simulink library "Contact_Forces_Lib"  (R2025a)
settings: Solver=ode45  StartTime=0.0  StopTime=10.0  RelTol=1e-3  EnableMultiTasking=on
undefined symbols (not defined in the file or in its folder): b_contact, custom_param_1, custom_param_2, Extr_Data_Ring, k_contact, l_cone, length_cylinder, length_tube, mu_kinetic, mu_static, pen_exponent, pen_full_damp_F, rad_s_cone, radius_cylinder, radius_tube, v_thr, X, Y, Z
libraries: nesl_utility x197, sm_lib x115, $bdroot x72, simulink x20, fl_lib x4
(part 12 of 12)

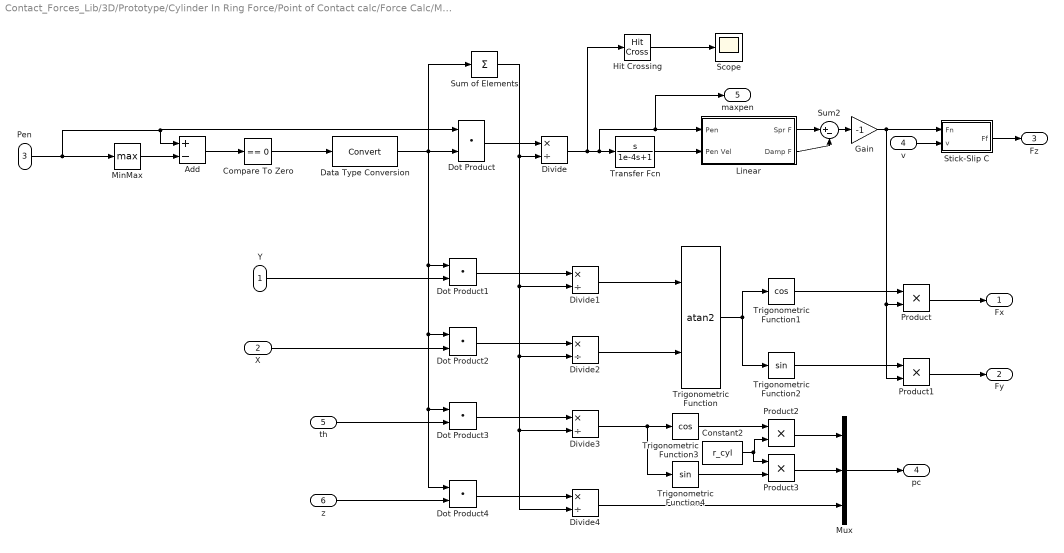
== system Contact_Forces_Lib/3D/Prototype/Cylinder In Ring Force/Point of Contact calc/Force Calc/MAX_SL ==
  Y : Inport
  X : Inport  Port=2
  Pen : Inport  Port=3
  v : Inport  Port=4
  th : Inport  Port=5
  z : Inport  Port=6
  Add : Sum  Inputs=+-
  Compare To Zero : simulink/Logic and Bit Operations/Compare To Zero  relop===  OutDataTypeStr=boolean  ZeroCross=off
  Constant2 : Constant  Value=r_cyl
  Data Type Conversion : DataTypeConversion  SaturateOnIntegerOverflow=off  RndMeth=Floor
  Divide{,1..4} (5 alike) : Product  Inputs=*/
  Dot Product{,1..4} (5 alike) : DotProduct  OutDataTypeStr=Inherit: Inherit via internal rule
  Gain : Gain  Gain=-1
  Hit Crossing : HitCross
  Linear : Subsystem  VariantControl=Linear  mask(Linear Force Law){k_pen=k_stiff, b_penvel=b_damp}
      mask prompts: k_pen "Contact Stiffness"; b_penvel "Contact Damping"
      mask help: Implements a contact force law as a linear spring damper. The damping force is applied only as the penetration depth increases.
      mask Help: web(which('Force_Laws.html'));
  MinMax : MinMax  Function=max  ZeroCross=off
  Mux : Mux  Inputs=3
  Product{,1..3} (4 alike) : Product
  Scope : Scope
      settings: DataLoggingVariableName=ScopeData3  DataLoggingSaveFormat=Array
  "Stick-Slip C " : Subsystem  VariantControl=Stick_Slip_C  mask(Stick-Slip Friction, Continuous){muk=mu_kinetic, mus=mu_static, vth=v_thr}
      mask prompts: muk "Coefficient of Kinetic Friction"; mus "Coefficient of Static Friction"; vth "Velocity Threshold"
      mask help: Implements a continuous stick-slip friction model. Smaller velocity threshold is closer to reality but results in a numerically stiffer system.
  Sum of Elements : Sum  Inputs=+
  Sum2 : Sum  Inputs=|+-
  Transfer Fcn : TransferFcn  Numerator=[1 0]  Denominator=[1e-4 1]
  Trigonometric Function : Trigonometry  Operator=atan2
  Trigonometric Function1 : Trigonometry  Operator=cos
  Trigonometric Function2 : Trigonometry
  Trigonometric Function3 : Trigonometry  Operator=cos
  Trigonometric Function4 : Trigonometry
  Fx : Outport  VectorParamsAs1DForOutWhenUnconnected=off
  Fy : Outport  Port=2  VectorParamsAs1DForOutWhenUnconnected=off
  Fz : Outport  Port=3  VectorParamsAs1DForOutWhenUnconnected=off
  pc : Outport  Port=4  VectorParamsAs1DForOutWhenUnconnected=off
  maxpen : Outport  Port=5  VectorParamsAs1DForOutWhenUnconnected=off
  wires:
  Trigonometric Function/1 -> Trigonometric Function2/1, Trigonometric Function1/1
  Linear/2(Damp F) -> Sum2/2
  Sum2/1 -> Gain/1
  Trigonometric Function2/1 -> Product1/1
  Linear/1(Spr F) -> Sum2/1
  Trigonometric Function1/1 -> Product/1
  Gain/1 -> "Stick-Slip C "/1(Fn), Product1/2, Product/2
  Transfer Fcn/1 -> Linear/2(Pen Vel)
  MinMax/1 -> Add/2
  Add/1 -> Compare To Zero/1
  Compare To Zero/1 -> Data Type Conversion/1
  Product/1 -> Fx/1
  Pen/1 -> Dot Product/1, Add/1, MinMax/1
  Product1/1 -> Fy/1
  Y/1 -> Dot Product1/2
  X/1 -> Dot Product2/2
  Data Type Conversion/1 -> Dot Product/2, Dot Product4/1, Dot Product3/1, Dot Product2/1, Dot Product1/1, Sum of Elements/1
  Dot Product/1 -> Divide/1
  Sum of Elements/1 -> Divide1/2, Divide4/2, Divide3/2, Divide2/2, Divide/2
  Divide/1 -> Hit Crossing/1, maxpen/1, Linear/1(Pen), Transfer Fcn/1
  Dot Product1/1 -> Divide1/1
  Dot Product2/1 -> Divide2/1
  Divide1/1 -> Trigonometric Function/1
  Divide2/1 -> Trigonometric Function/2
  Hit Crossing/1 -> Scope/1
  v/1 -> "Stick-Slip C "/2(v)
  Dot Product3/1 -> Divide3/1
  Dot Product4/1 -> Divide4/1
  th/1 -> Dot Product3/2
  z/1 -> Dot Product4/2
  Divide3/1 -> Trigonometric Function4/1, Trigonometric Function3/1
  Trigonometric Function3/1 -> Product2/1
  Trigonometric Function4/1 -> Product3/2
  Constant2/1 -> Product3/1, Product2/2
  Product2/1 -> Mux/1
  Product3/1 -> Mux/2
  Divide4/1 -> Mux/3
  "Stick-Slip C "/1(Ff) -> Fz/1
  Mux/1 -> pc/1

== system Contact_Forces_Lib/3D/Sphere to Cone Force/Forces/Ff/Relative vel at CP/Calculate vRelFace ==
  rSphtoCP sign : Inport
  azm : Inport  Port=2
  wxf : Inport  Port=3
  wyf : Inport  Port=4
  vzf : Inport  Port=5
  vrad : Inport  Port=6
  Gain : Gain  Gain=cosConeTh
  Gain{1..2,4..5} (4 alike) : Gain  Gain=-1
  Gain3 : Gain  Gain=sinConeTh
  Product : Product
  Product1 : Product
  Product2 : Product
  Sum : Sum
  Sum1 : Sum
  Sum3 : Sum
  Trigonometric Function3 : Trigonometry  Operator=cos
  Trigonometric Function4 : Trigonometry
  vRelFace : Outport  VectorParamsAs1DForOutWhenUnconnected=off
  wires:
  Gain4/1 -> Sum3/2  "vFaceTra"
  Gain5/1 -> Sum1/1
  Gain3/1 -> Gain5/1
  vzf/1 -> Gain3/1
  Gain/1 -> Sum1/2
  vrad/1 -> Gain/1
  Gain1/1 -> Product2/1
  Gain2/1 -> Sum/2  "wyCP"
  Trigonometric Function4/1 -> Product/1
  Product1/1 -> Gain2/1
  Sum3/1 -> vRelFace/1  "vRelFace"
  wyf/1 -> Product1/2
  Sum/1 -> Product2/2  "wxyzCP"
  rSphtoCP sign/1 -> Gain1/1
  Sum1/1 -> Gain4/1
  Product/1 -> Sum/1  "wxCP"
  wxf/1 -> Product/2
  Trigonometric Function3/1 -> Product1/1
  Product2/1 -> Sum3/1  "vFaceRot"
  azm/1 -> Trigonometric Function3/1, Trigonometric Function4/1

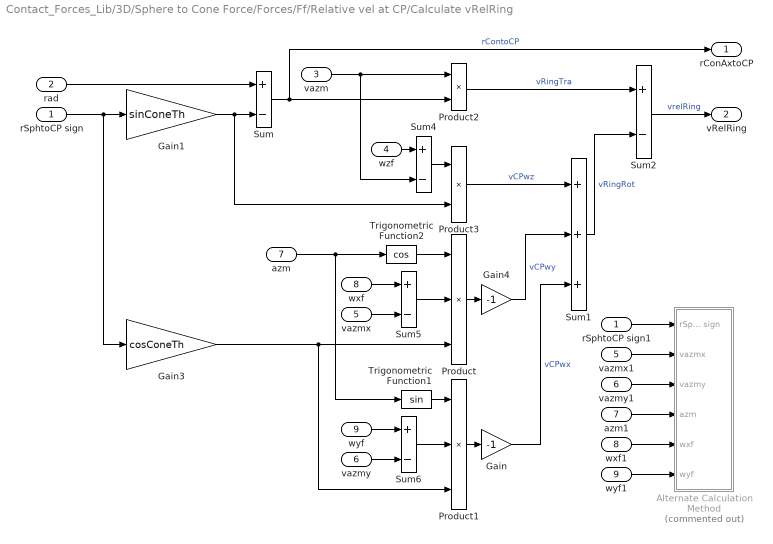
== system Contact_Forces_Lib/3D/Sphere to Cone Force/Forces/Ff/Relative vel at CP/Calculate vRelRing ==
  rSphtoCP sign : Inport
  rad : Inport  Port=2
  vazm : Inport  Port=3
  wzf : Inport  Port=4
  vazmx : Inport  Port=5
  vazmy : Inport  Port=6
  azm : Inport  Port=7
  wxf : Inport  Port=8
  wyf : Inport  Port=9
  Alternate Calculation Method : Subsystem  Commented=on
  Gain : Gain  Gain=-1
  Gain1 : Gain  Gain=sinConeTh
  Gain3 : Gain  Gain=cosConeTh
  Gain4 : Gain  Gain=-1
  Product : Product  Inputs=3
  Product1 : Product  Inputs=3
  Product2 : Product
  Product3 : Product
  Sum{,2,4..6} (5 alike) : Sum  Inputs=+-
  Sum1 : Sum  Inputs=+++
  Trigonometric Function1 : Trigonometry
  Trigonometric Function2 : Trigonometry  Operator=cos
  azm1 : InportShadow  Port=7
  rSphtoCP sign1 : InportShadow
  vazmx1 : InportShadow  Port=5
  vazmy1 : InportShadow  Port=6
  wxf1 : InportShadow  Port=8
  wyf1 : InportShadow  Port=9
  rConAxtoCP : Outport  VectorParamsAs1DForOutWhenUnconnected=off
  vRelRing : Outport  Port=2  VectorParamsAs1DForOutWhenUnconnected=off
  wires:
  wyf1/1 -> Alternate Calculation Method/6(wyf)
  wxf1/1 -> Alternate Calculation Method/5(wxf)
  azm1/1 -> Alternate Calculation Method/4(azm)
  vazmy1/1 -> Alternate Calculation Method/3(vazmy)
  vazmx1/1 -> Alternate Calculation Method/2(vazmx)
  rSphtoCP sign1/1 -> Alternate Calculation Method/1(rSphtoCP sign)
  Gain4/1 -> Sum1/2  "vCPwy"
  Sum6/1 -> Product1/2
  vazmy/1 -> Sum6/2
  wyf/1 -> Sum6/1
  vazmx/1 -> Sum5/2
  wxf/1 -> Sum5/1
  Product3/1 -> Sum1/1  "vCPwz"
  Gain3/1 -> Product1/3, Product/3
  Gain/1 -> Sum1/3  "vCPwx"
  Product1/1 -> Gain/1
  Trigonometric Function1/1 -> Product1/1
  Sum5/1 -> Product/2
  azm/1 -> Trigonometric Function1/1, Trigonometric Function2/1
  Product/1 -> Gain4/1
  Trigonometric Function2/1 -> Product/1
  Gain1/1 -> Sum/2, Product3/2
  rSphtoCP sign/1 -> Gain3/1, Gain1/1
  rad/1 -> Sum/1
  wzf/1 -> Sum4/1
  vazm/1 -> Product2/1, Sum4/2
  Product2/1 -> Sum2/1  "vRingTra"
  Sum/1 -> rConAxtoCP/1, Product2/2  "rContoCP"
  Sum2/1 -> vRelRing/1  "vrelRing"
  Sum1/1 -> Sum2/2  "vRingRot"
  Sum4/1 -> Product3/1

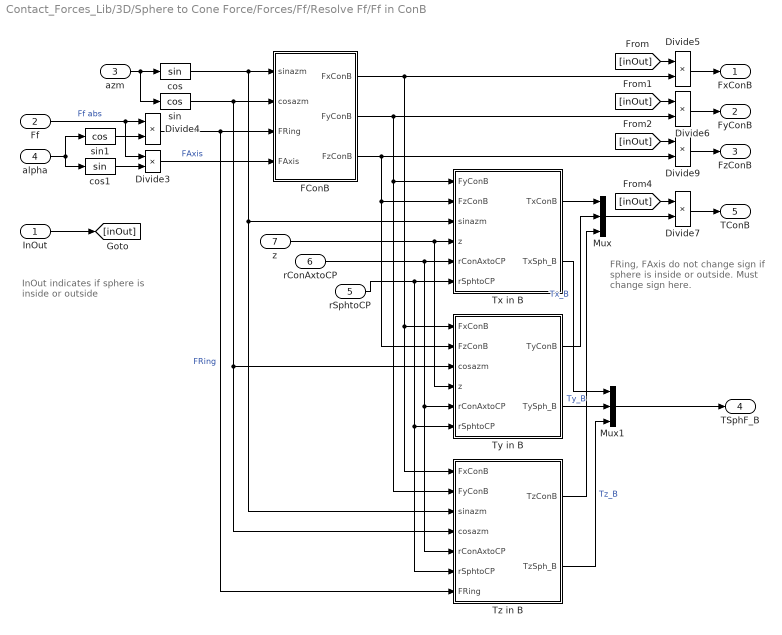
== system Contact_Forces_Lib/3D/Sphere to Cone Force/Forces/Ff/Resolve Ff/Ff in ConB ==
  note: InOut indicates if sphere is inside or outside
  note: FRing, FAxis do not change sign if sphere is inside or outside. Must change sign here.
  InOut : Inport
  Ff : Inport  Port=2
  azm : Inport  Port=3
  alpha : Inport  Port=4
  rSphtoCP : Inport  Port=5
  rConAxtoCP : Inport  Port=6
  z : Inport  Port=7
  Divide{3..7,9} (6 alike) : Product  Inputs=**
  FConB : Subsystem
  Mux : Mux  Inputs=3
  Mux1 : Mux  Inputs=3
  Tx in B : Subsystem
  Ty in B : Subsystem
  Tz in B : Subsystem
  cos : Trigonometry
  cos1 : Trigonometry
  sin : Trigonometry  Operator=cos
  sin1 : Trigonometry  Operator=cos
  FxConB : Outport  VectorParamsAs1DForOutWhenUnconnected=off
  FyConB : Outport  Port=2  VectorParamsAs1DForOutWhenUnconnected=off
  FzConB : Outport  Port=3  VectorParamsAs1DForOutWhenUnconnected=off
  TSphF_B : Outport  Port=4  VectorParamsAs1DForOutWhenUnconnected=off
  TConB : Outport  Port=5  VectorParamsAs1DForOutWhenUnconnected=off
  wires:
  FConB/2(FyConB) -> Divide6/2, Tz in B/2(FyConB), Tx in B/1(FyConB)
  Mux1/1 -> TSphF_B/1
  Divide3/1 -> FConB/4(FAxis)  "FAxis"
  FConB/1(FxConB) -> Ty in B/1(FxConB), Tz in B/1(FxConB), Divide5/2
  FConB/3(FzConB) -> Divide9/2, Ty in B/2(FzConB), Tx in B/2(FzConB)
  Divide4/1 -> FConB/3(FRing), Tz in B/7(FRing)  "FRing"
  Mux/1 -> Divide7/2
  Ff/1 -> Divide4/1, Divide3/1  "Ff abs"
  alpha/1 -> cos1/1, sin1/1
  cos1/1 -> Divide3/2
  sin/1 -> FConB/2(cosazm), Ty in B/3(cosazm), Tz in B/4(cosazm)
  azm/1 -> cos/1, sin/1
  cos/1 -> FConB/1(sinazm), Tz in B/3(sinazm), Tx in B/3(sinazm)
  sin1/1 -> Divide4/2
  rConAxtoCP/1 -> Tx in B/5(rConAxtoCP), Ty in B/5(rConAxtoCP), Tz in B/5(rConAxtoCP)
  rSphtoCP/1 -> Ty in B/6(rSphtoCP), Tz in B/6(rSphtoCP), Tx in B/6(rSphtoCP)
  z/1 -> Ty in B/4(z), Tx in B/4(z)
  Tx in B/1(TxConB) -> Mux/1
  Ty in B/1(TyConB) -> Mux/2
  Tx in B/2(TxSph_B) -> Mux1/1  "Tx_B"
  Ty in B/2(TySph_B) -> Mux1/2  "Ty_B"
  InOut/1 -> [inOut]
  Divide9/1 -> FzConB/1
  Divide5/1 -> FxConB/1
  Divide6/1 -> FyConB/1
  [inOut] -> Divide5/1
  [inOut] -> Divide6/1
  [inOut] -> Divide9/1
  Tz in B/1(TzConB) -> Mux/3
  Tz in B/2(TzSph_B) -> Mux1/3  "Tz_B"
  [inOut] -> Divide7/1
  Divide7/1 -> TConB/1

== system Contact_Forces_Lib/3D/Sphere to Cone Force/Forces/Ff/Resolve Ff/Ff in SphF ==
  FxConB : Inport
  FyConB : Inport  Port=2
  FzConB : Inport  Port=3
  TSphF_B : Inport  Port=4
  R : Inport  Port=5
  Demux : Demux  Outputs=3
  Divide1 : Product  Inputs=/*  Multiplication=Matrix(*)
  Divide3 : Product  Inputs=/*  Multiplication=Matrix(*)
  Gain1 : Gain  Gain=-1
  Mux1 : Mux  Inputs=3
  FySphF : Outport  VectorParamsAs1DForOutWhenUnconnected=off
  FxSphF : Outport  Port=2  VectorParamsAs1DForOutWhenUnconnected=off
  FzSphF : Outport  Port=3  VectorParamsAs1DForOutWhenUnconnected=off
  TSphF : Outport  Port=4  VectorParamsAs1DForOutWhenUnconnected=off
  wires:
  TSphF_B/1 -> Divide1/2
  Demux/3 -> FzSphF/1
  Demux/2 -> FySphF/1
  Demux/1 -> FxSphF/1
  FzConB/1 -> Mux1/3
  FxConB/1 -> Mux1/1
  FyConB/1 -> Mux1/2
  Gain1/1 -> Demux/1
  Mux1/1 -> Divide3/2
  Divide3/1 -> Gain1/1
  R/1 -> Divide3/1, Divide1/1
  Divide1/1 -> TSphF/1

== system Contact_Forces_Lib/3D/Sphere to Tube Force/Forces/Ff/Relative vel at CP/Calculate vRelAxis ==
  rSphtoCP sign : Inport
  wxf : Inport  Port=2
  vzf : Inport  Port=3
  azm : Inport  Port=4
  wyf : Inport  Port=5
  " " : Gain  Gain=-1
  Product4 : Product
  Product5 : Product
  Product6 : Product
  Sum4 : Sum  Inputs=+-
  Sum5 : Sum
  Trigonometric Function1 : Trigonometry
  Trigonometric Function2 : Trigonometry  Operator=cos
  vRelAxis : Outport  VectorParamsAs1DForOutWhenUnconnected=off
  wires:
  " "/1 -> Sum5/2  "wCPy"
  Product6/1 -> " "/1
  wxf/1 -> Product5/1
  Product5/1 -> Sum5/1  "wCPx"
  Trigonometric Function2/1 -> Product6/1
  Sum4/1 -> vRelAxis/1  "vRelAxis"
  vzf/1 -> Sum4/1  "vAxisTra"
  Sum5/1 -> Product4/2  "wCP"
  azm/1 -> Trigonometric Function2/1, Trigonometric Function1/1
  wyf/1 -> Product6/2
  Product4/1 -> Sum4/2  "vAxisRot"
  Trigonometric Function1/1 -> Product5/2
  rSphtoCP sign/1 -> Product4/1

== system Contact_Forces_Lib/3D/Sphere to Tube Force/Forces/Ff/Relative vel at CP/Calculate vRelRing ==
  rad : Inport
  vazm : Inport  Port=2
  wzf : Inport  Port=3
  rSphtoCP sign : Inport  Port=4
  Product1 : Product
  Product2 : Product
  Sum : Sum  Inputs=+-
  Sum1 : Sum  Inputs=+-
  Sum2 : Sum  Inputs=+-
  rCyltoCP : Outport  VectorParamsAs1DForOutWhenUnconnected=off
  vRelRing : Outport  Port=2  VectorParamsAs1DForOutWhenUnconnected=off
  wires:
  Product1/1 -> Sum2/2  "vRingRot"
  Sum2/1 -> vRelRing/1  "vrelRing"
  Sum/1 -> rCyltoCP/1, Product2/2  "rCyltoCP"
  Product2/1 -> Sum2/1  "vRingTra"
  vazm/1 -> Product2/1, Sum1/2
  wzf/1 -> Sum1/1
  rad/1 -> Sum/1
  rSphtoCP sign/1 -> Product1/2, Sum/2
  Sum1/1 -> Product1/1

== system Contact_Forces_Lib/3D/Sphere to Tube Force/Forces/Ff/Resolve Ff/Ff in SphF ==
  FxTubB : Inport
  FyTubB : Inport  Port=2
  FzTubB : Inport  Port=3
  TSphF_B : Inport  Port=4
  R : Inport  Port=5
  Demux : Demux  Outputs=3
  Divide1 : Product  Inputs=/*  Multiplication=Matrix(*)
  Divide3 : Product  Inputs=/*  Multiplication=Matrix(*)
  Gain1 : Gain  Gain=-1
  Mux1 : Mux  Inputs=3
  FySphF : Outport  VectorParamsAs1DForOutWhenUnconnected=off
  FxSphF : Outport  Port=2  VectorParamsAs1DForOutWhenUnconnected=off
  FzSphF : Outport  Port=3  VectorParamsAs1DForOutWhenUnconnected=off
  TSphF : Outport  Port=4  VectorParamsAs1DForOutWhenUnconnected=off
  wires:
  Divide1/1 -> TSphF/1
  R/1 -> Divide1/1, Divide3/1
  Divide3/1 -> Gain1/1
  Mux1/1 -> Divide3/2
  Gain1/1 -> Demux/1
  FyTubB/1 -> Mux1/2
  FxTubB/1 -> Mux1/1
  FzTubB/1 -> Mux1/3
  Demux/1 -> FxSphF/1
  Demux/2 -> FySphF/1
  Demux/3 -> FzSphF/1
  TSphF_B/1 -> Divide1/2

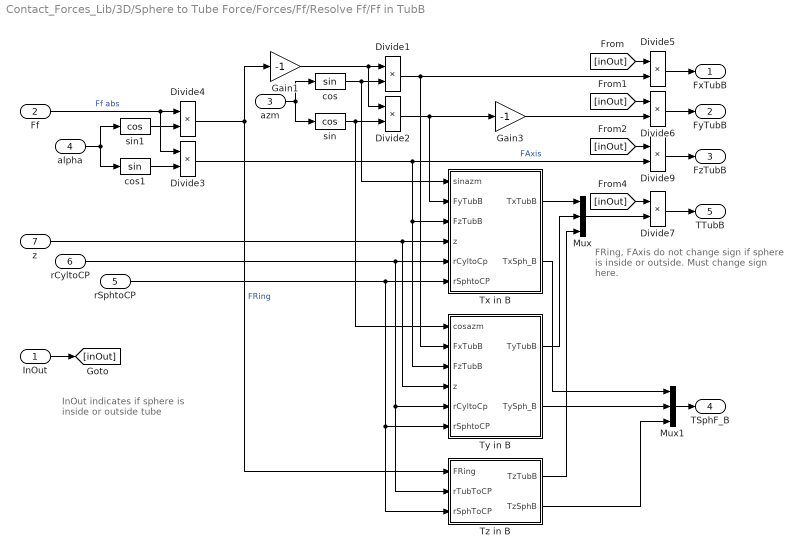
== system Contact_Forces_Lib/3D/Sphere to Tube Force/Forces/Ff/Resolve Ff/Ff in TubB ==
  note: FRing, FAxis do not change sign if sphere is inside or outside. Must change sign here.
  note: InOut indicates if sphere is inside or outside tube
  InOut : Inport
  Ff : Inport  Port=2
  azm : Inport  Port=3
  alpha : Inport  Port=4
  rSphtoCP : Inport  Port=5
  rCyltoCP : Inport  Port=6
  z : Inport  Port=7
  Divide{1..7,9} (8 alike) : Product  Inputs=**
  Gain1 : Gain  Gain=-1
  Gain3 : Gain  Gain=-1
  Mux : Mux  Inputs=3
  Mux1 : Mux  Inputs=3
  Tx in B : Subsystem
  Ty in B : Subsystem
  Tz in B : Subsystem
  cos : Trigonometry
  cos1 : Trigonometry
  sin : Trigonometry  Operator=cos
  sin1 : Trigonometry  Operator=cos
  FxTubB : Outport  VectorParamsAs1DForOutWhenUnconnected=off
  FyTubB : Outport  Port=2  VectorParamsAs1DForOutWhenUnconnected=off
  FzTubB : Outport  Port=3  VectorParamsAs1DForOutWhenUnconnected=off
  TSphF_B : Outport  Port=4  VectorParamsAs1DForOutWhenUnconnected=off
  TTubB : Outport  Port=5  VectorParamsAs1DForOutWhenUnconnected=off
  wires:
  Divide7/1 -> TTubB/1
  Gain3/1 -> Divide6/2
  [inOut] -> Divide7/1
  Tz in B/2(TzSphB) -> Mux1/3
  Tz in B/1(TzTubB) -> Mux/3
  [inOut] -> Divide9/1
  [inOut] -> Divide6/1
  [inOut] -> Divide5/1
  Divide6/1 -> FyTubB/1
  Divide5/1 -> FxTubB/1
  Divide9/1 -> FzTubB/1
  InOut/1 -> [inOut]
  Gain1/1 -> Divide2/1, Divide1/1
  Ty in B/2(TySph_B) -> Mux1/2
  Tx in B/2(TxSph_B) -> Mux1/1
  Ty in B/1(TyTubB) -> Mux/2
  Divide1/1 -> Divide5/2, Ty in B/2(FxTubB)
  Tx in B/1(TxTubB) -> Mux/1
  z/1 -> Tx in B/4(z), Ty in B/4(z)
  rSphtoCP/1 -> Tz in B/3(rSphToCP), Ty in B/6(rSphtoCP), Tx in B/6(rSphtoCP)
  rCyltoCP/1 -> Tx in B/5(rCyltoCp), Ty in B/5(rCyltoCp), Tz in B/2(rTubToCP)
  sin1/1 -> Divide4/2
  cos/1 -> Divide1/2, Tx in B/1(sinazm)
  azm/1 -> cos/1, sin/1
  Divide2/1 -> Tx in B/2(FyTubB), Gain3/1
  sin/1 -> Ty in B/1(cosazm), Divide2/2
  cos1/1 -> Divide3/2
  alpha/1 -> sin1/1, cos1/1
  Ff/1 -> Divide4/1, Divide3/1  "Ff abs"
  Mux1/1 -> TSphF_B/1
  Mux/1 -> Divide7/2
  Divide4/1 -> Gain1/1, Tz in B/1(FRing)  "FRing"
  Divide3/1 -> Ty in B/3(FzTubB), Tx in B/3(FzTubB), Divide9/2  "FAxis"

== system Contact_Forces_Lib/3D/Sphere to Tube Force Enabled/Forces/Ff/Relative vel at CP/Calculate vRelAxis ==
  rSphtoCP sign : Inport
  wxf : Inport  Port=2
  vzf : Inport  Port=3
  azm : Inport  Port=4
  wyf : Inport  Port=5
  " " : Gain  Gain=-1
  Product4 : Product
  Product5 : Product
  Product6 : Product
  Sum4 : Sum  Inputs=+-
  Sum5 : Sum
  Trigonometric Function1 : Trigonometry
  Trigonometric Function2 : Trigonometry  Operator=cos
  vRelAxis : Outport  VectorParamsAs1DForOutWhenUnconnected=off
  wires:
  " "/1 -> Sum5/2  "wCPy"
  Product6/1 -> " "/1
  wxf/1 -> Product5/1
  Product5/1 -> Sum5/1  "wCPx"
  Trigonometric Function2/1 -> Product6/1
  Sum4/1 -> vRelAxis/1  "vRelAxis"
  vzf/1 -> Sum4/1  "vAxisTra"
  Sum5/1 -> Product4/2  "wCP"
  azm/1 -> Trigonometric Function2/1, Trigonometric Function1/1
  wyf/1 -> Product6/2
  Product4/1 -> Sum4/2  "vAxisRot"
  Trigonometric Function1/1 -> Product5/2
  rSphtoCP sign/1 -> Product4/1

== system Contact_Forces_Lib/3D/Sphere to Tube Force Enabled/Forces/Ff/Relative vel at CP/Calculate vRelRing ==
  rad : Inport
  vazm : Inport  Port=2
  wzf : Inport  Port=3
  rSphtoCP sign : Inport  Port=4
  Product1 : Product
  Product2 : Product
  Sum : Sum  Inputs=+-
  Sum1 : Sum  Inputs=+-
  Sum2 : Sum  Inputs=+-
  rCyltoCP : Outport  VectorParamsAs1DForOutWhenUnconnected=off
  vRelRing : Outport  Port=2  VectorParamsAs1DForOutWhenUnconnected=off
  wires:
  Product1/1 -> Sum2/2  "vRingRot"
  Sum2/1 -> vRelRing/1  "vrelRing"
  Sum/1 -> rCyltoCP/1, Product2/2  "rCyltoCP"
  Product2/1 -> Sum2/1  "vRingTra"
  vazm/1 -> Product2/1, Sum1/2
  wzf/1 -> Sum1/1
  rad/1 -> Sum/1
  rSphtoCP sign/1 -> Product1/2, Sum/2
  Sum1/1 -> Product1/1

== system Contact_Forces_Lib/3D/Sphere to Tube Force Enabled/Forces/Ff/Resolve Ff/Ff in SphF ==
  FxTubB : Inport
  FyTubB : Inport  Port=2
  FzTubB : Inport  Port=3
  TSphF_B : Inport  Port=4
  R : Inport  Port=5
  Demux : Demux  Outputs=3
  Divide1 : Product  Inputs=/*  Multiplication=Matrix(*)
  Divide3 : Product  Inputs=/*  Multiplication=Matrix(*)
  Gain1 : Gain  Gain=-1
  Mux1 : Mux  Inputs=3
  FySphF : Outport  VectorParamsAs1DForOutWhenUnconnected=off
  FxSphF : Outport  Port=2  VectorParamsAs1DForOutWhenUnconnected=off
  FzSphF : Outport  Port=3  VectorParamsAs1DForOutWhenUnconnected=off
  TSphF : Outport  Port=4  VectorParamsAs1DForOutWhenUnconnected=off
  wires:
  Divide1/1 -> TSphF/1
  R/1 -> Divide1/1, Divide3/1
  Divide3/1 -> Gain1/1
  Mux1/1 -> Divide3/2
  Gain1/1 -> Demux/1
  FyTubB/1 -> Mux1/2
  FxTubB/1 -> Mux1/1
  FzTubB/1 -> Mux1/3
  Demux/1 -> FxSphF/1
  Demux/2 -> FySphF/1
  Demux/3 -> FzSphF/1
  TSphF_B/1 -> Divide1/2

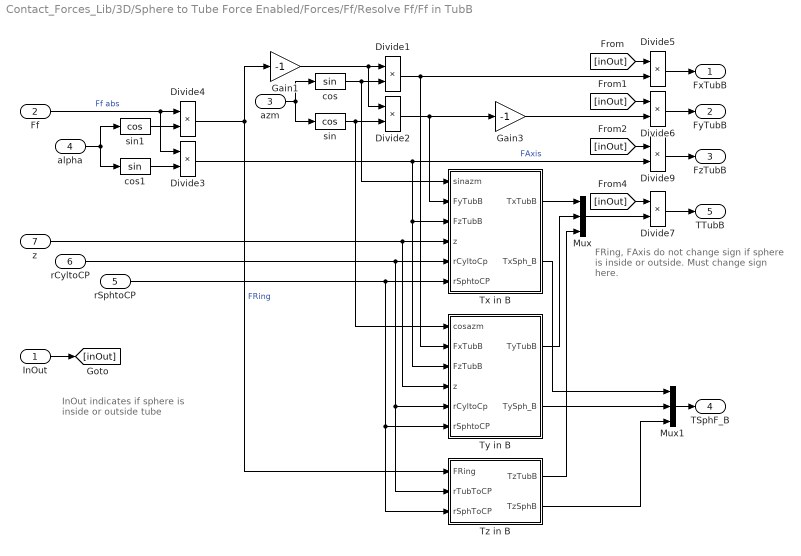
== system Contact_Forces_Lib/3D/Sphere to Tube Force Enabled/Forces/Ff/Resolve Ff/Ff in TubB ==
  note: FRing, FAxis do not change sign if sphere is inside or outside. Must change sign here.
  note: InOut indicates if sphere is inside or outside tube
  InOut : Inport
  Ff : Inport  Port=2
  azm : Inport  Port=3
  alpha : Inport  Port=4
  rSphtoCP : Inport  Port=5
  rCyltoCP : Inport  Port=6
  z : Inport  Port=7
  Divide{1..7,9} (8 alike) : Product  Inputs=**
  Gain1 : Gain  Gain=-1
  Gain3 : Gain  Gain=-1
  Mux : Mux  Inputs=3
  Mux1 : Mux  Inputs=3
  Tx in B : Subsystem
  Ty in B : Subsystem
  Tz in B : Subsystem
  cos : Trigonometry
  cos1 : Trigonometry
  sin : Trigonometry  Operator=cos
  sin1 : Trigonometry  Operator=cos
  FxTubB : Outport  VectorParamsAs1DForOutWhenUnconnected=off
  FyTubB : Outport  Port=2  VectorParamsAs1DForOutWhenUnconnected=off
  FzTubB : Outport  Port=3  VectorParamsAs1DForOutWhenUnconnected=off
  TSphF_B : Outport  Port=4  VectorParamsAs1DForOutWhenUnconnected=off
  TTubB : Outport  Port=5  VectorParamsAs1DForOutWhenUnconnected=off
  wires:
  Divide7/1 -> TTubB/1
  Gain3/1 -> Divide6/2
  [inOut] -> Divide7/1
  Tz in B/2(TzSphB) -> Mux1/3
  Tz in B/1(TzTubB) -> Mux/3
  [inOut] -> Divide9/1
  [inOut] -> Divide6/1
  [inOut] -> Divide5/1
  Divide6/1 -> FyTubB/1
  Divide5/1 -> FxTubB/1
  Divide9/1 -> FzTubB/1
  InOut/1 -> [inOut]
  Gain1/1 -> Divide2/1, Divide1/1
  Ty in B/2(TySph_B) -> Mux1/2
  Tx in B/2(TxSph_B) -> Mux1/1
  Ty in B/1(TyTubB) -> Mux/2
  Divide1/1 -> Divide5/2, Ty in B/2(FxTubB)
  Tx in B/1(TxTubB) -> Mux/1
  z/1 -> Tx in B/4(z), Ty in B/4(z)
  rSphtoCP/1 -> Tz in B/3(rSphToCP), Ty in B/6(rSphtoCP), Tx in B/6(rSphtoCP)
  rCyltoCP/1 -> Tx in B/5(rCyltoCp), Ty in B/5(rCyltoCp), Tz in B/2(rTubToCP)
  sin1/1 -> Divide4/2
  cos/1 -> Divide1/2, Tx in B/1(sinazm)
  azm/1 -> cos/1, sin/1
  Divide2/1 -> Tx in B/2(FyTubB), Gain3/1
  sin/1 -> Ty in B/1(cosazm), Divide2/2
  cos1/1 -> Divide3/2
  alpha/1 -> sin1/1, cos1/1
  Ff/1 -> Divide4/1, Divide3/1  "Ff abs"
  Mux1/1 -> TSphF_B/1
  Mux/1 -> Divide7/2
  Divide4/1 -> Gain1/1, Tz in B/1(FRing)  "FRing"
  Divide3/1 -> Ty in B/3(FzTubB), Tx in B/3(FzTubB), Divide9/2  "FAxis"

== system Contact_Forces_Lib/3D/Prototype/Cone in Ring Force/Point of Contact calc/Force Calc/Computing Force from nonzero penetration points/For Each Subsystem1 ==
  In1 : Inport  Partition=on  PartitionDimension=1  PartitionWidth=1  PartitionOffset=0
  For Each : ForEach  DisableCoverage=on
  Transfer Fcn1 : TransferFcn  Numerator=[1 0]  Denominator=[1e-4 1]
  Out1 : Outport  ConcatenationDimension=1  VectorParamsAs1DForOutWhenUnconnected=off
  wires:
  In1/1 -> Transfer Fcn1/1
  Transfer Fcn1/1 -> Out1/1

== system Contact_Forces_Lib/3D/Prototype/Cone in Ring Force/Point of Contact calc/Force Calc/Computing Force from nonzero penetration points/For Iterator Subsystem ==
  Pen : Inport
  X : Inport  Port=2
  Y : Inport  Port=3
  Penv : Inport  Port=4
  Delay : Delay  DelayLength=1  InitialCondition=0
  Delay1 : Delay  DelayLength=1  InitialCondition=0
  For Iterator : ForIterator  ResetStates=reset  IterationSource=external
  Gain : Gain  Gain=-1
  Linear : Subsystem  VariantControl=Linear  mask(Linear Force Law){k_pen=1e6, b_penvel=1e4}
      mask prompts: k_pen "Contact Stiffness"; b_penvel "Contact Damping"
      mask help: Implements a contact force law as a linear spring damper. The damping force is applied only as the penetration depth increases.
      mask Help: web(which('Force_Laws.html'));
  Product : Product
  Product1 : Product
  Selector{,1..3} (4 alike) : Selector  IndexOptions=Index vector (port)  Indices=[1 3]  OutputSizes=1
  Sum : Sum  Inputs=|++
  Sum1 : Sum  Inputs=|++
  Sum2 : Sum  Inputs=|+-
  Trigonometric Function : Trigonometry  Operator=atan2
  Trigonometric Function1 : Trigonometry  Operator=cos
  Trigonometric Function2 : Trigonometry
  Width : Width
  Fx : Outport  VectorParamsAs1DForOutWhenUnconnected=off
  Fy : Outport  Port=2  VectorParamsAs1DForOutWhenUnconnected=off
  wires:
  Trigonometric Function/1 -> Trigonometric Function2/1, Trigonometric Function1/1
  Linear/2(Damp F) -> Sum2/2
  Sum2/1 -> Gain/1
  Trigonometric Function2/1 -> Product1/1
  Linear/1(Spr F) -> Sum2/1
  Trigonometric Function1/1 -> Product/1
  Gain/1 -> Product/2, Product1/2
  Product1/1 -> Sum1/1
  Product/1 -> Sum/1
  Width/1 -> For Iterator/1
  Pen/1 -> Selector/1, Width/1
  Selector/1 -> Linear/1(Pen)
  For Iterator/1 -> Selector2/2, Selector3/2, Selector/2, Selector1/2
  Y/1 -> Selector1/1
  X/1 -> Selector2/1
  Selector1/1 -> Trigonometric Function/1
  Selector2/1 -> Trigonometric Function/2
  Penv/1 -> Selector3/1
  Sum/1 -> Delay/1, Fx/1
  Delay/1 -> Sum/2
  Sum1/1 -> Delay1/1, Fy/1
  Delay1/1 -> Sum1/2
  Selector3/1 -> Linear/2(Pen Vel)

== system Contact_Forces_Lib/3D/Prototype/Cone in Ring Force/Point of Contact calc/Force Calc/Computing Force from nonzero penetration points/Linear1 ==
  Pen : Inport
  Pen Vel : Inport  Port=2
  Abs : Abs  ZeroCross=off  SaturateOnIntegerOverflow=off
  Gain1 : Gain  Gain=k_pen  Multiplication=Matrix(K*u)  SaturateOnIntegerOverflow=on  OutDataTypeStr=Inherit: Same as input  ParamDataTypeStr=Inherit: Same as input
  Gain2 : Gain  Gain=-b_penvel  Multiplication=Matrix(K*u)  SaturateOnIntegerOverflow=on  OutDataTypeStr=Inherit: Same as input  ParamDataTypeStr=Inherit: Same as input
  Product : Product  RndMeth=Zero
  Saturation : Saturate  UpperLimit=Inf  LowerLimit=0  ZeroCross=off
  Sign : Signum  ZeroCross=off
  Spr F : Outport  VectorParamsAs1DForOutWhenUnconnected=off
  Damp F : Outport  Port=2  VectorParamsAs1DForOutWhenUnconnected=off
  wires:
  Gain1/1 -> Spr F/1  "Stiffness_Force"
  Gain2/1 -> Product/2  "Damping_Force"
  Pen Vel/1 -> Saturation/1  "Pen Vel"
  Sign/1 -> Abs/1
  Product/1 -> Damp F/1  "Damping_Force"
  Abs/1 -> Product/1  "Damping_Force_Enable"
  Pen/1 -> Gain1/1, Sign/1  "Penetration"
  Saturation/1 -> Gain2/1

== system Contact_Forces_Lib/3D/Prototype/Cone in Ring Force/Point of Contact calc/Force Calc/MAX_ML/Linear ==
  Pen : Inport
  Pen Vel : Inport  Port=2
  Abs : Abs  ZeroCross=off  SaturateOnIntegerOverflow=off
  Gain1 : Gain  Gain=k_pen  Multiplication=Matrix(K*u)  SaturateOnIntegerOverflow=on  OutDataTypeStr=Inherit: Same as input  ParamDataTypeStr=Inherit: Same as input
  Gain2 : Gain  Gain=-b_penvel  Multiplication=Matrix(K*u)  SaturateOnIntegerOverflow=on  OutDataTypeStr=Inherit: Same as input  ParamDataTypeStr=Inherit: Same as input
  Product : Product  RndMeth=Zero
  Saturation : Saturate  UpperLimit=Inf  LowerLimit=0  ZeroCross=off
  Sign : Signum  ZeroCross=off
  Spr F : Outport  VectorParamsAs1DForOutWhenUnconnected=off
  Damp F : Outport  Port=2  VectorParamsAs1DForOutWhenUnconnected=off
  wires:
  Saturation/1 -> Gain2/1
  Pen/1 -> Sign/1, Gain1/1  "Penetration"
  Abs/1 -> Product/1  "Damping_Force_Enable"
  Product/1 -> Damp F/1  "Damping_Force"
  Sign/1 -> Abs/1
  Pen Vel/1 -> Saturation/1  "Pen Vel"
  Gain2/1 -> Product/2  "Damping_Force"
  Gain1/1 -> Spr F/1  "Stiffness_Force"

== system Contact_Forces_Lib/3D/Prototype/Cone in Ring Force/Point of Contact calc/Force Calc/MAX_SL/Linear ==
  Pen : Inport
  Pen Vel : Inport  Port=2
  Abs : Abs  ZeroCross=off  SaturateOnIntegerOverflow=off
  Gain1 : Gain  Gain=k_pen  Multiplication=Matrix(K*u)  SaturateOnIntegerOverflow=on  OutDataTypeStr=Inherit: Same as input  ParamDataTypeStr=Inherit: Same as input
  Gain2 : Gain  Gain=-b_penvel  Multiplication=Matrix(K*u)  SaturateOnIntegerOverflow=on  OutDataTypeStr=Inherit: Same as input  ParamDataTypeStr=Inherit: Same as input
  Product : Product  RndMeth=Zero
  Saturation : Saturate  UpperLimit=Inf  LowerLimit=0  ZeroCross=off
  Sign : Signum  ZeroCross=off
  Spr F : Outport  VectorParamsAs1DForOutWhenUnconnected=off
  Damp F : Outport  Port=2  VectorParamsAs1DForOutWhenUnconnected=off
  wires:
  Gain1/1 -> Spr F/1  "Stiffness_Force"
  Gain2/1 -> Product/2  "Damping_Force"
  Pen Vel/1 -> Saturation/1  "Pen Vel"
  Sign/1 -> Abs/1
  Product/1 -> Damp F/1  "Damping_Force"
  Abs/1 -> Product/1  "Damping_Force_Enable"
  Pen/1 -> Gain1/1, Sign/1  "Penetration"
  Saturation/1 -> Gain2/1

== system Contact_Forces_Lib/3D/Prototype/Cylinder In Ring Force/Point of Contact calc/Force Calc/Computing Force from nonzero penetration points/For Each Subsystem1 ==
  In1 : Inport  Partition=on  PartitionDimension=1  PartitionWidth=1  PartitionOffset=0
  For Each : ForEach  DisableCoverage=on
  Transfer Fcn1 : TransferFcn  Numerator=[1 0]  Denominator=[1e-4 1]
  Out1 : Outport  ConcatenationDimension=1  VectorParamsAs1DForOutWhenUnconnected=off
  wires:
  In1/1 -> Transfer Fcn1/1
  Transfer Fcn1/1 -> Out1/1

== system Contact_Forces_Lib/3D/Prototype/Cylinder In Ring Force/Point of Contact calc/Force Calc/Computing Force from nonzero penetration points/For Iterator Subsystem ==
  Pen : Inport
  X : Inport  Port=2
  Y : Inport  Port=3
  Penv : Inport  Port=4
  Delay : Delay  DelayLength=1  InitialCondition=0
  Delay1 : Delay  DelayLength=1  InitialCondition=0
  For Iterator : ForIterator  ResetStates=reset  IterationSource=external
  Gain : Gain  Gain=-1
  Linear : Subsystem  VariantControl=Linear  mask(Linear Force Law){k_pen=1e6, b_penvel=1e4}
      mask prompts: k_pen "Contact Stiffness"; b_penvel "Contact Damping"
      mask help: Implements a contact force law as a linear spring damper. The damping force is applied only as the penetration depth increases.
      mask Help: web(which('Force_Laws.html'));
  Product : Product
  Product1 : Product
  Selector{,1..3} (4 alike) : Selector  IndexOptions=Index vector (port)  Indices=[1 3]  OutputSizes=1
  Sum : Sum  Inputs=|++
  Sum1 : Sum  Inputs=|++
  Sum2 : Sum  Inputs=|+-
  Trigonometric Function : Trigonometry  Operator=atan2
  Trigonometric Function1 : Trigonometry  Operator=cos
  Trigonometric Function2 : Trigonometry
  Width : Width
  Fx : Outport  VectorParamsAs1DForOutWhenUnconnected=off
  Fy : Outport  Port=2  VectorParamsAs1DForOutWhenUnconnected=off
  wires:
  Trigonometric Function/1 -> Trigonometric Function2/1, Trigonometric Function1/1
  Linear/2(Damp F) -> Sum2/2
  Sum2/1 -> Gain/1
  Trigonometric Function2/1 -> Product1/1
  Linear/1(Spr F) -> Sum2/1
  Trigonometric Function1/1 -> Product/1
  Gain/1 -> Product/2, Product1/2
  Product1/1 -> Sum1/1
  Product/1 -> Sum/1
  Width/1 -> For Iterator/1
  Pen/1 -> Selector/1, Width/1
  Selector/1 -> Linear/1(Pen)
  For Iterator/1 -> Selector2/2, Selector3/2, Selector/2, Selector1/2
  Y/1 -> Selector1/1
  X/1 -> Selector2/1
  Selector1/1 -> Trigonometric Function/1
  Selector2/1 -> Trigonometric Function/2
  Penv/1 -> Selector3/1
  Sum/1 -> Delay/1, Fx/1
  Delay/1 -> Sum/2
  Sum1/1 -> Delay1/1, Fy/1
  Delay1/1 -> Sum1/2
  Selector3/1 -> Linear/2(Pen Vel)

== system Contact_Forces_Lib/3D/Prototype/Cylinder In Ring Force/Point of Contact calc/Force Calc/Computing Force from nonzero penetration points/Linear1 ==
  Pen : Inport
  Pen Vel : Inport  Port=2
  Abs : Abs  ZeroCross=off  SaturateOnIntegerOverflow=off
  Gain1 : Gain  Gain=k_pen  Multiplication=Matrix(K*u)  SaturateOnIntegerOverflow=on  OutDataTypeStr=Inherit: Same as input  ParamDataTypeStr=Inherit: Same as input
  Gain2 : Gain  Gain=-b_penvel  Multiplication=Matrix(K*u)  SaturateOnIntegerOverflow=on  OutDataTypeStr=Inherit: Same as input  ParamDataTypeStr=Inherit: Same as input
  Product : Product  RndMeth=Zero
  Saturation : Saturate  UpperLimit=Inf  LowerLimit=0  ZeroCross=off
  Sign : Signum  ZeroCross=off
  Spr F : Outport  VectorParamsAs1DForOutWhenUnconnected=off
  Damp F : Outport  Port=2  VectorParamsAs1DForOutWhenUnconnected=off
  wires:
  Gain1/1 -> Spr F/1  "Stiffness_Force"
  Gain2/1 -> Product/2  "Damping_Force"
  Pen Vel/1 -> Saturation/1  "Pen Vel"
  Sign/1 -> Abs/1
  Product/1 -> Damp F/1  "Damping_Force"
  Abs/1 -> Product/1  "Damping_Force_Enable"
  Pen/1 -> Gain1/1, Sign/1  "Penetration"
  Saturation/1 -> Gain2/1

== system Contact_Forces_Lib/3D/Prototype/Cylinder In Ring Force/Point of Contact calc/Force Calc/MAX_ML/Linear ==
  Pen : Inport
  Pen Vel : Inport  Port=2
  Abs : Abs  ZeroCross=off  SaturateOnIntegerOverflow=off
  Gain1 : Gain  Gain=k_pen  Multiplication=Matrix(K*u)  SaturateOnIntegerOverflow=on  OutDataTypeStr=Inherit: Same as input  ParamDataTypeStr=Inherit: Same as input
  Gain2 : Gain  Gain=-b_penvel  Multiplication=Matrix(K*u)  SaturateOnIntegerOverflow=on  OutDataTypeStr=Inherit: Same as input  ParamDataTypeStr=Inherit: Same as input
  Product : Product  RndMeth=Zero
  Saturation : Saturate  UpperLimit=Inf  LowerLimit=0  ZeroCross=off
  Sign : Signum  ZeroCross=off
  Spr F : Outport  VectorParamsAs1DForOutWhenUnconnected=off
  Damp F : Outport  Port=2  VectorParamsAs1DForOutWhenUnconnected=off
  wires:
  Saturation/1 -> Gain2/1
  Pen/1 -> Sign/1, Gain1/1  "Penetration"
  Abs/1 -> Product/1  "Damping_Force_Enable"
  Product/1 -> Damp F/1  "Damping_Force"
  Sign/1 -> Abs/1
  Pen Vel/1 -> Saturation/1  "Pen Vel"
  Gain2/1 -> Product/2  "Damping_Force"
  Gain1/1 -> Spr F/1  "Stiffness_Force"

== system Contact_Forces_Lib/3D/Prototype/Cylinder In Ring Force/Point of Contact calc/Force Calc/MAX_SL/Linear ==
  Pen : Inport
  Pen Vel : Inport  Port=2
  Abs : Abs  ZeroCross=off  SaturateOnIntegerOverflow=off
  Gain1 : Gain  Gain=k_pen  Multiplication=Matrix(K*u)  SaturateOnIntegerOverflow=on  OutDataTypeStr=Inherit: Same as input  ParamDataTypeStr=Inherit: Same as input
  Gain2 : Gain  Gain=-b_penvel  Multiplication=Matrix(K*u)  SaturateOnIntegerOverflow=on  OutDataTypeStr=Inherit: Same as input  ParamDataTypeStr=Inherit: Same as input
  Product : Product  RndMeth=Zero
  Saturation : Saturate  UpperLimit=Inf  LowerLimit=0  ZeroCross=off
  Sign : Signum  ZeroCross=off
  Spr F : Outport  VectorParamsAs1DForOutWhenUnconnected=off
  Damp F : Outport  Port=2  VectorParamsAs1DForOutWhenUnconnected=off
  wires:
  Gain1/1 -> Spr F/1  "Stiffness_Force"
  Gain2/1 -> Product/2  "Damping_Force"
  Pen Vel/1 -> Saturation/1  "Pen Vel"
  Sign/1 -> Abs/1
  Product/1 -> Damp F/1  "Damping_Force"
  Abs/1 -> Product/1  "Damping_Force_Enable"
  Pen/1 -> Gain1/1, Sign/1  "Penetration"
  Saturation/1 -> Gain2/1

== system Contact_Forces_Lib/3D/Prototype/Cylinder In Ring Force/Point of Contact calc/Force Calc/MAX_SL/Stick-Slip C  ==
  Fn : Inport
  v : Inport  Port=2
  Coefficient of Friction vs Velocity : Lookup_n-D  NumberOfTableDimensions=1  BreakpointsForDimension1=[-3 -1.5 -1 1 1.5 3]*vth  Table="[-muk -muk -mus mus  muk muk]"  InternalRulePriority=Speed
  Gain2 : Gain  Multiplication=Matrix(K*u)  SaturateOnIntegerOverflow=on  OutDataTypeStr=Inherit: Same as input  ParamDataTypeStr=Inherit: Same as input
  Product : Product  RndMeth=Zero
  Ff : Outport  VectorParamsAs1DForOutWhenUnconnected=off
  wires:
  Fn/1 -> Product/2  "Normal_Force"
  Coefficient of Friction vs Velocity/1 -> Product/1
  v/1 -> Coefficient of Friction vs Velocity/1  "Velocity"
  Product/1 -> Gain2/1
  Gain2/1 -> Ff/1  "Friction_Force"

== system Contact_Forces_Lib/3D/Sphere to Cone Force/Forces/Ff/Relative vel at CP/Calculate vRelRing/Alternate Calculation Method ==
  rSphtoCP sign : Inport
  vazmx : Inport  Port=2
  vazmy : Inport  Port=3
  azm : Inport  Port=4
  wxf : Inport  Port=5
  wyf : Inport  Port=6
  Sum3 : Sum  Inputs=+-
  Sum7 : Sum  Inputs=+-
  Terminator : Terminator
  Terminator1 : Terminator
  Trigonometric Function3 : Trigonometry  Operator=cos
  Trigonometric Function4 : Trigonometry
  vCPinRingWx : Subsystem
  vCPinRingWy : Subsystem
  wires:
  Sum7/1 -> vCPinRingWy/3(wy)
  vazmy/1 -> Sum7/2
  wyf/1 -> Sum7/1
  Trigonometric Function4/1 -> vCPinRingWy/1(sinazm)
  Sum3/1 -> vCPinRingWx/3(wx)
  azm/1 -> Trigonometric Function3/1, Trigonometric Function4/1
  vazmx/1 -> Sum3/2
  Trigonometric Function3/1 -> vCPinRingWx/1(cosazm)
  wxf/1 -> Sum3/1
  rSphtoCP sign/1 -> vCPinRingWx/2(rSphtoCP sign), vCPinRingWy/2(rSphtoCP sign)
  vCPinRingWy/1(vCPinRingWy) -> Terminator1/1
  vCPinRingWx/1(vCPinRingWx) -> Terminator/1

== system Contact_Forces_Lib/3D/Sphere to Cone Force/Forces/Ff/Resolve Ff/Ff in ConB/FConB ==
  sinazm : Inport
  cosazm : Inport  Port=2
  FRing : Inport  Port=3
  FAxis : Inport  Port=4
  Divide{1..4} (4 alike) : Product  Inputs=**
  Gain : Gain  Gain=cosConeTh
  Gain1 : Gain  Gain=sinConeTh
  Gain2 : Gain  Gain=-1
  Gain3 : Gain  Gain=-1
  Gain4 : Gain  Gain=-1
  Sum : Sum
  Sum1 : Sum
  FxConB : Outport  VectorParamsAs1DForOutWhenUnconnected=off
  FyConB : Outport  Port=2  VectorParamsAs1DForOutWhenUnconnected=off
  FzConB : Outport  Port=3  VectorParamsAs1DForOutWhenUnconnected=off
  wires:
  Gain4/1 -> Sum1/1
  Divide1/1 -> Gain4/1
  Sum1/1 -> FxConB/1  "FxConB"
  Gain3/1 -> Sum1/2
  Divide4/1 -> Gain3/1
  Sum/1 -> FyConB/1  "FyConB"
  Gain2/1 -> Sum/2
  Divide3/1 -> Gain2/1
  Gain/1 -> Divide4/2, Divide3/2
  Gain1/1 -> FzConB/1  "FzConB"
  sinazm/1 -> Divide1/2, Divide3/1
  cosazm/1 -> Divide2/2, Divide4/1
  Divide2/1 -> Sum/1
  FRing/1 -> Divide1/1, Divide2/1
  FAxis/1 -> Gain/1, Gain1/1

== system Contact_Forces_Lib/3D/Sphere to Cone Force/Forces/Ff/Resolve Ff/Ff in ConB/Tx in B ==
  FyConB : Inport
  FzConB : Inport  Port=2
  sinazm : Inport  Port=3
  z : Inport  Port=4
  rConAxtoCP : Inport  Port=5
  rSphtoCP : Inport  Port=6
  Divide1 : Product  Inputs=***
  Divide{2..5} (4 alike) : Product  Inputs=**
  Gain : Gain  Gain=cosConeTh
  Gain1 : Gain  Gain=sinConeTh
  Gain2 : Gain  Gain=-1
  Gain3 : Gain  Gain=-1
  Sum : Sum
  Sum1 : Sum
  TxConB : Outport  VectorParamsAs1DForOutWhenUnconnected=off
  TxSph_B : Outport  Port=2  VectorParamsAs1DForOutWhenUnconnected=off
  wires:
  Gain2/1 -> Sum1/2
  Sum1/1 -> TxSph_B/1
  Gain3/1 -> Sum/2
  rConAxtoCP/1 -> Divide1/3
  sinazm/1 -> Divide1/1, Divide5/1
  Divide4/1 -> Gain2/1
  Divide3/1 -> Sum1/1
  FyConB/1 -> Divide4/2, Divide2/1
  Gain/1 -> Divide4/1
  Divide5/1 -> Divide3/2
  Gain1/1 -> Divide5/2
  Divide2/1 -> Gain3/1
  z/1 -> Divide2/2
  rSphtoCP/1 -> Gain/1, Gain1/1
  FzConB/1 -> Divide1/2, Divide3/1
  Divide1/1 -> Sum/1
  Sum/1 -> TxConB/1

== system Contact_Forces_Lib/3D/Sphere to Cone Force/Forces/Ff/Resolve Ff/Ff in ConB/Ty in B ==
  FxConB : Inport
  FzConB : Inport  Port=2
  cosazm : Inport  Port=3
  z : Inport  Port=4
  rConAxtoCP : Inport  Port=5
  rSphtoCP : Inport  Port=6
  Divide1 : Product  Inputs=***
  Divide2 : Product  Inputs=**
  Divide4 : Product  Inputs=***
  Divide5 : Product  Inputs=**
  Gain : Gain  Gain=cosConeTh
  Gain1 : Gain  Gain=sinConeTh
  Gain2 : Gain  Gain=-1
  Gain3 : Gain  Gain=-1
  Sum : Sum
  Sum1 : Sum
  TyConB : Outport  VectorParamsAs1DForOutWhenUnconnected=off
  TySph_B : Outport  Port=2  VectorParamsAs1DForOutWhenUnconnected=off
  wires:
  Gain/1 -> Divide5/2
  Gain3/1 -> Sum/1
  FzConB/1 -> Divide4/3, Divide1/1
  Sum/1 -> TyConB/1
  Divide1/1 -> Gain3/1
  FxConB/1 -> Divide5/1, Divide2/1
  rSphtoCP/1 -> Gain1/1, Gain/1
  z/1 -> Divide2/2
  Gain1/1 -> Divide4/1
  cosazm/1 -> Divide4/2, Divide1/2
  Divide4/1 -> Gain2/1
  Divide5/1 -> Sum1/1
  Gain2/1 -> Sum1/2
  Sum1/1 -> TySph_B/1
  rConAxtoCP/1 -> Divide1/3
  Divide2/1 -> Sum/2

== system Contact_Forces_Lib/3D/Sphere to Cone Force/Forces/Ff/Resolve Ff/Ff in ConB/Tz in B ==
  FxConB : Inport
  FyConB : Inport  Port=2
  sinazm : Inport  Port=3
  cosazm : Inport  Port=4
  rConAxtoCP : Inport  Port=5
  rSphtoCP : Inport  Port=6
  FRing : Inport  Port=7
  Divide2 : Product  Inputs=**
  Divide4 : Product  Inputs=***
  Divide5 : Product  Inputs=***
  Gain1 : Gain  Gain=sinConeTh
  Gain4 : Gain  Gain=-1
  Sum1 : Sum
  TzConB : Outport  VectorParamsAs1DForOutWhenUnconnected=off
  TzSph_B : Outport  Port=2  VectorParamsAs1DForOutWhenUnconnected=off
  wires:
  FRing/1 -> Divide2/2
  rConAxtoCP/1 -> Divide2/1
  sinazm/1 -> Divide5/2
  Sum1/1 -> TzSph_B/1
  Divide4/1 -> Sum1/2
  Gain4/1 -> Sum1/1
  cosazm/1 -> Divide4/2
  Gain1/1 -> Divide5/3, Divide4/1
  rSphtoCP/1 -> Gain1/1
  FxConB/1 -> Divide5/1
  Divide2/1 -> TzConB/1
  Divide5/1 -> Gain4/1
  FyConB/1 -> Divide4/3

== system Contact_Forces_Lib/3D/Sphere to Tube Force/Forces/Ff/Resolve Ff/Ff in TubB/Tx in B ==
  sinazm : Inport
  FyTubB : Inport  Port=2
  FzTubB : Inport  Port=3
  z : Inport  Port=4
  rCyltoCp : Inport  Port=5
  rSphtoCP : Inport  Port=6
  Divide{1..2,5..6} (4 alike) : Product  Inputs=**
  Sum : Sum
  TxTubB : Outport  VectorParamsAs1DForOutWhenUnconnected=off
  TxSph_B : Outport  Port=2  VectorParamsAs1DForOutWhenUnconnected=off
  wires:
  Sum/1 -> TxTubB/1
  Divide1/1 -> TxSph_B/1
  FyTubB/1 -> Divide6/1
  Divide5/1 -> Divide2/1, Divide1/2
  rSphtoCP/1 -> Divide1/1
  rCyltoCp/1 -> Divide2/2
  FzTubB/1 -> Divide5/1
  sinazm/1 -> Divide5/2
  z/1 -> Divide6/2
  Divide6/1 -> Sum/2
  Divide2/1 -> Sum/1

== system Contact_Forces_Lib/3D/Sphere to Tube Force/Forces/Ff/Resolve Ff/Ff in TubB/Ty in B ==
  cosazm : Inport
  FxTubB : Inport  Port=2
  FzTubB : Inport  Port=3
  z : Inport  Port=4
  rCyltoCp : Inport  Port=5
  rSphtoCP : Inport  Port=6
  Divide{1..2,5..6} (4 alike) : Product  Inputs=**
  Gain2 : Gain  Gain=-1
  Sum : Sum
  TyTubB : Outport  VectorParamsAs1DForOutWhenUnconnected=off
  TySph_B : Outport  Port=2  VectorParamsAs1DForOutWhenUnconnected=off
  wires:
  Sum/1 -> TyTubB/1
  Gain2/1 -> Divide5/1
  Divide2/1 -> Sum/1
  Divide6/1 -> Sum/2
  z/1 -> Divide6/2
  cosazm/1 -> Divide5/2
  FzTubB/1 -> Gain2/1
  rCyltoCp/1 -> Divide2/2
  rSphtoCP/1 -> Divide1/1
  Divide5/1 -> Divide2/1, Divide1/2
  FxTubB/1 -> Divide6/1
  Divide1/1 -> TySph_B/1

== system Contact_Forces_Lib/3D/Sphere to Tube Force/Forces/Ff/Resolve Ff/Ff in TubB/Tz in B ==
  FRing : Inport
  rTubToCP : Inport  Port=2
  rSphToCP : Inport  Port=3
  Divide7 : Product  Inputs=**
  Divide8 : Product  Inputs=**
  TzTubB : Outport  VectorParamsAs1DForOutWhenUnconnected=off
  TzSphB : Outport  Port=2  VectorParamsAs1DForOutWhenUnconnected=off
  wires:
  FRing/1 -> Divide8/1, Divide7/1
  rSphToCP/1 -> Divide7/2
  rTubToCP/1 -> Divide8/2
  Divide7/1 -> TzSphB/1
  Divide8/1 -> TzTubB/1  "TzTubB"

== system Contact_Forces_Lib/3D/Sphere to Tube Force Enabled/Forces/Ff/Resolve Ff/Ff in TubB/Tx in B ==
  sinazm : Inport
  FyTubB : Inport  Port=2
  FzTubB : Inport  Port=3
  z : Inport  Port=4
  rCyltoCp : Inport  Port=5
  rSphtoCP : Inport  Port=6
  Divide{1..2,5..6} (4 alike) : Product  Inputs=**
  Sum : Sum
  TxTubB : Outport  VectorParamsAs1DForOutWhenUnconnected=off
  TxSph_B : Outport  Port=2  VectorParamsAs1DForOutWhenUnconnected=off
  wires:
  Sum/1 -> TxTubB/1
  Divide1/1 -> TxSph_B/1
  FyTubB/1 -> Divide6/1
  Divide5/1 -> Divide2/1, Divide1/2
  rSphtoCP/1 -> Divide1/1
  rCyltoCp/1 -> Divide2/2
  FzTubB/1 -> Divide5/1
  sinazm/1 -> Divide5/2
  z/1 -> Divide6/2
  Divide6/1 -> Sum/2
  Divide2/1 -> Sum/1

== system Contact_Forces_Lib/3D/Sphere to Tube Force Enabled/Forces/Ff/Resolve Ff/Ff in TubB/Ty in B ==
  cosazm : Inport
  FxTubB : Inport  Port=2
  FzTubB : Inport  Port=3
  z : Inport  Port=4
  rCyltoCp : Inport  Port=5
  rSphtoCP : Inport  Port=6
  Divide{1..2,5..6} (4 alike) : Product  Inputs=**
  Gain2 : Gain  Gain=-1
  Sum : Sum
  TyTubB : Outport  VectorParamsAs1DForOutWhenUnconnected=off
  TySph_B : Outport  Port=2  VectorParamsAs1DForOutWhenUnconnected=off
  wires:
  Sum/1 -> TyTubB/1
  Gain2/1 -> Divide5/1
  Divide2/1 -> Sum/1
  Divide6/1 -> Sum/2
  z/1 -> Divide6/2
  cosazm/1 -> Divide5/2
  FzTubB/1 -> Gain2/1
  rCyltoCp/1 -> Divide2/2
  rSphtoCP/1 -> Divide1/1
  Divide5/1 -> Divide2/1, Divide1/2
  FxTubB/1 -> Divide6/1
  Divide1/1 -> TySph_B/1

== system Contact_Forces_Lib/3D/Sphere to Tube Force Enabled/Forces/Ff/Resolve Ff/Ff in TubB/Tz in B ==
  FRing : Inport
  rTubToCP : Inport  Port=2
  rSphToCP : Inport  Port=3
  Divide7 : Product  Inputs=**
  Divide8 : Product  Inputs=**
  TzTubB : Outport  VectorParamsAs1DForOutWhenUnconnected=off
  TzSphB : Outport  Port=2  VectorParamsAs1DForOutWhenUnconnected=off
  wires:
  FRing/1 -> Divide8/1, Divide7/1
  rSphToCP/1 -> Divide7/2
  rTubToCP/1 -> Divide8/2
  Divide7/1 -> TzSphB/1
  Divide8/1 -> TzTubB/1  "TzTubB"

== system Contact_Forces_Lib/3D/Prototype/Cone in Ring Force/Point of Contact calc/Force Calc/Computing Force from nonzero penetration points/For Iterator Subsystem/Linear ==
  Pen : Inport
  Pen Vel : Inport  Port=2
  Abs : Abs  ZeroCross=off  SaturateOnIntegerOverflow=off
  Gain1 : Gain  Gain=k_pen  Multiplication=Matrix(K*u)  SaturateOnIntegerOverflow=on  OutDataTypeStr=Inherit: Same as input  ParamDataTypeStr=Inherit: Same as input
  Gain2 : Gain  Gain=-b_penvel  Multiplication=Matrix(K*u)  SaturateOnIntegerOverflow=on  OutDataTypeStr=Inherit: Same as input  ParamDataTypeStr=Inherit: Same as input
  Product : Product  RndMeth=Zero
  Saturation : Saturate  UpperLimit=Inf  LowerLimit=0  ZeroCross=off
  Sign : Signum  ZeroCross=off
  Spr F : Outport  VectorParamsAs1DForOutWhenUnconnected=off
  Damp F : Outport  Port=2  VectorParamsAs1DForOutWhenUnconnected=off
  wires:
  Gain1/1 -> Spr F/1  "Stiffness_Force"
  Gain2/1 -> Product/2  "Damping_Force"
  Pen Vel/1 -> Saturation/1  "Pen Vel"
  Sign/1 -> Abs/1
  Product/1 -> Damp F/1  "Damping_Force"
  Abs/1 -> Product/1  "Damping_Force_Enable"
  Pen/1 -> Gain1/1, Sign/1  "Penetration"
  Saturation/1 -> Gain2/1

== system Contact_Forces_Lib/3D/Prototype/Cylinder In Ring Force/Point of Contact calc/Force Calc/Computing Force from nonzero penetration points/For Iterator Subsystem/Linear ==
  Pen : Inport
  Pen Vel : Inport  Port=2
  Abs : Abs  ZeroCross=off  SaturateOnIntegerOverflow=off
  Gain1 : Gain  Gain=k_pen  Multiplication=Matrix(K*u)  SaturateOnIntegerOverflow=on  OutDataTypeStr=Inherit: Same as input  ParamDataTypeStr=Inherit: Same as input
  Gain2 : Gain  Gain=-b_penvel  Multiplication=Matrix(K*u)  SaturateOnIntegerOverflow=on  OutDataTypeStr=Inherit: Same as input  ParamDataTypeStr=Inherit: Same as input
  Product : Product  RndMeth=Zero
  Saturation : Saturate  UpperLimit=Inf  LowerLimit=0  ZeroCross=off
  Sign : Signum  ZeroCross=off
  Spr F : Outport  VectorParamsAs1DForOutWhenUnconnected=off
  Damp F : Outport  Port=2  VectorParamsAs1DForOutWhenUnconnected=off
  wires:
  Gain1/1 -> Spr F/1  "Stiffness_Force"
  Gain2/1 -> Product/2  "Damping_Force"
  Pen Vel/1 -> Saturation/1  "Pen Vel"
  Sign/1 -> Abs/1
  Product/1 -> Damp F/1  "Damping_Force"
  Abs/1 -> Product/1  "Damping_Force_Enable"
  Pen/1 -> Gain1/1, Sign/1  "Penetration"
  Saturation/1 -> Gain2/1

== system Contact_Forces_Lib/3D/Sphere to Cone Force/Forces/Ff/Relative vel at CP/Calculate vRelRing/Alternate Calculation Method/vCPinRingWx ==
  cosazm : Inport
  rSphtoCP sign : Inport  Port=2
  wx : Inport  Port=3
  Constant : Constant  Value=pi/2
  Constant1 : Constant  Value=sinConeTh
  Constant2 : Constant  Value=cosConeTh
  Gain : Gain  Gain=-1
  Math Function : Math  Operator=square  SignedPower=on
  Math Function1 : Math  Operator=square  SignedPower=on
  Product : Product  Inputs=4
  Product1 : Product  Inputs=3
  Product2 : Product
  Sqrt : Sqrt
  Subtract : Sum  Inputs=+-
  Subtract1 : Sum
  Trigonometric Function : Trigonometry  Operator=cos
  Trigonometric Function1 : Trigonometry  Operator=atan2
  vCPinRingWx : Outport  VectorParamsAs1DForOutWhenUnconnected=off
  wires:
  Gain/1 -> vCPinRingWx/1
  wx/1 -> Product/1
  rSphtoCP sign/1 -> Product1/1, Product2/1
  Constant2/1 -> Product2/2
  Constant1/1 -> Product1/2
  Math Function1/1 -> Subtract1/1
  Math Function/1 -> Subtract1/2
  cosazm/1 -> Product/4, Product1/3
  Subtract1/1 -> Sqrt/1
  Sqrt/1 -> Product/2
  Product1/1 -> Trigonometric Function1/2, Math Function/1  "Rx"
  Product2/1 -> Trigonometric Function1/1, Math Function1/1  "Rz"
  Trigonometric Function1/1 -> Subtract/2
  Constant/1 -> Subtract/1
  Subtract/1 -> Trigonometric Function/1
  Trigonometric Function/1 -> Product/3
  Product/1 -> Gain/1

== system Contact_Forces_Lib/3D/Sphere to Cone Force/Forces/Ff/Relative vel at CP/Calculate vRelRing/Alternate Calculation Method/vCPinRingWy ==
  sinazm : Inport
  rSphtoCP sign : Inport  Port=2
  wy : Inport  Port=3
  Constant : Constant  Value=pi/2
  Constant1 : Constant  Value=sinConeTh
  Constant2 : Constant  Value=cosConeTh
  Gain : Gain  Gain=-1
  Math Function : Math  Operator=square  SignedPower=on
  Math Function1 : Math  Operator=square  SignedPower=on
  Product : Product  Inputs=4
  Product1 : Product  Inputs=3
  Product2 : Product
  Sqrt : Sqrt
  Subtract : Sum  Inputs=+-
  Subtract1 : Sum
  Trigonometric Function : Trigonometry  Operator=cos
  Trigonometric Function1 : Trigonometry  Operator=atan2
  vCPinRingWy : Outport  VectorParamsAs1DForOutWhenUnconnected=off
  wires:
  Product/1 -> Gain/1
  Trigonometric Function/1 -> Product/3
  Subtract/1 -> Trigonometric Function/1
  Constant/1 -> Subtract/1
  Trigonometric Function1/1 -> Subtract/2
  Product2/1 -> Math Function1/1, Trigonometric Function1/1  "Rz"
  Product1/1 -> Math Function/1, Trigonometric Function1/2  "Rx"
  Sqrt/1 -> Product/2
  Subtract1/1 -> Sqrt/1
  sinazm/1 -> Product1/3, Product/4
  Math Function/1 -> Subtract1/2
  Math Function1/1 -> Subtract1/1
  Constant1/1 -> Product1/2
  Constant2/1 -> Product2/2
  rSphtoCP sign/1 -> Product2/1, Product1/1
  wy/1 -> Product/1
  Gain/1 -> vCPinRingWy/1

== matlab function Contact_Forces_Lib/3D/Prototype/Cylinder In Ring Force/Point of Contact calc/Force Calc/MAX_ML/MATLAB Function ==
  data: pen input; x input; y input; xc output; yc output; penc output; ind output
function [xc, yc, penc,ind] = fcn(pen, x, y)
%#codegen
[val,ind] = max(pen);

% if val == 0
%     penc = 0;
%     xc = 0;
%     yc = 0; 
% else
    penc = pen(ind);
    xc = x(ind);
    yc = y(ind);
% end

== matlab function Contact_Forces_Lib/3D/Prototype/Cone in Ring Force/Point of Contact calc/Force Calc/MAX_ML/MATLAB Function ==
  data: pen input; x input; y input; xc output; yc output; penc output; ind output
function [xc, yc, penc,ind] = fcn(pen, x, y)
%#codegen
[val,ind] = max(pen);

% if val == 0
%     penc = 0;
%     xc = 0;
%     yc = 0; 
% else
    penc = pen(ind);
    xc = x(ind);
    yc = y(ind);
% end
